simulink model "HorizontalBaseline"  (R2026b)
settings: Solver=FixedStepDiscrete  StopTime=inf  FixedStep=Official.Step
PostLoadFcn:
  | run(fullfile(fileparts(get_param('StampFly_IMU400','FileName')),'config','startup.m'));
InitFcn:
  | init_imu_flight;
undefined symbols (not defined in the file): Official
libraries: slpidlib x7, simulink x4, mspfiltlib x1
(part 1 of 5)
settings Model: SILPILModeSetting=veronly  Creator=tyasukaw  LastModifiedBy=tyasukaw
settings SolverCC: AutoInsertRateTranBlk=on
settings OptimizationCC: DifferentSizesBufferReuse=on  EfficientTunableParamExpr=on  EnhancedBackFolding=on  MaxStackSize=64  OptimizationCustomize=off  OptimizeBlockOrder=speed  PassReuseOutputArgsAs=Individual arguments  RemoveInternalMemoryZeroInit=on  RemoveRootLevelIOMemoryZeroInit=on
settings DebuggingCC: ParameterTunabilityLossMsg=error
settings HardwareCC: ProdHWDeviceType=ARM Compatible->ARM Cortex  ProdLargestAtomicFloat=Double  ProdLargestAtomicInteger=Long
settings SFSimCC: MATLABDynamicMemAlloc=off
settings RTWCC: BuildConfiguration=Faster Runs  DataTypeReplacement=CDataTypesFixedWidth  Description=Embedded Coder  HardwareBoard=ESP32-S3 Series (Arduino Compatible)  SystemTargetFile=ert.tlc  TLCOptions="-aInlineSetEventsForThisBaseRateFcn=TLC_FALSE -aSuppressMultiTaskScheduler=TLC_FALSE  -aRateBasedStepFcn=0"  TemplateMakefile=ert_default_tmf  Toolchain=ESP32
settings CodeAppCC: ForceParamTrailComments=on  IgnoreCustomStorageClasses=off  InsertBlockDesc=on  OperatorAnnotations=on  SFDataObjDesc=on  SimulinkDataObjDesc=on
settings ERTTargetCC: CombineSignalStateStructs=on  ExtModeAutomaticAllocSize=off  ExtModeIntrfLevel=Level2 - Open  ExtModeMexFile=ext_xcp  ExtModeStaticAlloc=on  MaxIdInt16=INT16_MAX  MaxIdInt32=INT32_MAX  MaxIdInt64=INT64_MAX  MaxIdInt8=INT8_MAX  MaxIdUint16=UINT16_MAX  MaxIdUint32=UINT32_MAX  MaxIdUint64=UINT64_MAX  MaxIdUint8=UINT8_MAX  MinIdInt16=INT16_MIN  MinIdInt32=INT32_MIN  MinIdInt64=INT64_MIN  MinIdInt8=INT8_MIN  SupportContinuousTime=on  SupportVariableSizeSignals=on

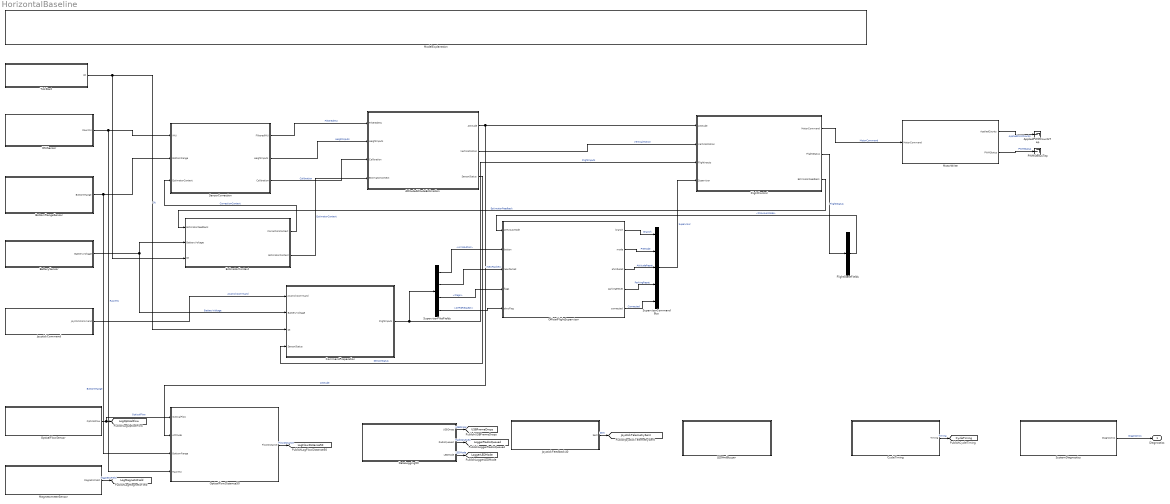
== system HorizontalBaseline ==
  AppliedPWMCountsTap : Terminator
      settings: Description=AppliedPWMCountsTap：使用しない観測出力をここで終端します。接続された制御信号を変更しません。
  AttitudeAltitudeEstimation : Subsystem  Description=IMU Filter で姿勢・補正済み角速度、MATLAB Function の AltitudeKalman で高度・鉛直速度を推定します。状態フラグと推定診断をまとめ、ログ用 Goto をこの階層から公開します。
      mask help: IMU Filter で姿勢・補正済み角速度、MATLAB Function の AltitudeKalman で高度・鉛直速度を推定します。状態フラグと推定診断をまとめ、ログ用 Goto をこの階層から公開します。
      mask Display: disp('AttitudeAltitudeEstimation');port_label('input',1,'FilteredIMU');port_label('input',2,'HeightInputs');port_label('input',3,'Calibration');port_label('input',4,'EstimatorContext');port_label('output',1,'Attitude');port_label('output',2,'VerticalMotion');port_label('output',3,'SensorStatus');
  BatterySensor : Subsystem  Description=電池電圧 [V] と読み出し有効性を取得します。I2C 使用中は前回値を保持し、ReadValid=0 を公開します。
      mask help: 電池電圧 [V] と読み出し有効性を取得します。I2C 使用中は前回値を保持し、ReadValid=0 を公開します。
      mask Display: disp('BatterySensor');port_label('output',1,'BatteryVoltage');
  BottomRangeSensor : Subsystem  Description=下向き ToF の初期化完了後は Mode に依存せず取得します。距離 [mm] と Fresh を BottomRange バスへまとめ、Status と診断は Goto で公開します。Fresh は 400 Hz の読み出しではなく新しい測定結果の到着を示します。前方センサーは未使用です。
      mask help: 下向き ToF の初期化完了後は Mode に依存せず取得します。距離 [mm] と Fresh を BottomRange バスへまとめ、Status と診断は Goto で公開します。Fresh は 400 Hz の読み出しではなく新しい測定結果の到着を示します。前方センサーは未使用です。
      mask Display: disp('BottomRangeSensor');port_label('output',1,'BottomRange');
  CommandPreparation : Subsystem  Description=操縦指令、電池電圧、実測 dt、センサーフラグを名前付きバスへまとめます。Stateflow と飛行制御へ同じ入力を渡し、ログ用の観測も公開します。
      mask help: 操縦指令、電池電圧、実測 dt、センサーフラグを名前付きバスへまとめます。Stateflow と飛行制御へ同じ入力を渡し、ログ用の観測も公開します。
      mask Display: disp('CommandPreparation');port_label('input',1,'JoystickCommand');port_label('input',2,'BatteryVoltage');port_label('input',3,'Dt');port_label('input',4,'SensorStatus');port_label('output',1,'FlightInputs');
  CycleTiming : Subsystem  Description=ログとモーター適用後の処理時間・周期間隔を観測します。制御値を変更せず、計測位置を信号依存で固定します。
      mask help: ログとモーター適用後の処理時間・周期間隔を観測します。制御値を変更せず、計測位置を信号依存で固定します。
      mask Display: disp('CycleTiming');port_label('output',1,'Timing');
  DataLogging50 : Subsystem  Description=生センサー・推定・制御・追加センサーを名前付き From で取得し、50 Hz の SFI8/SFIX/SFIY ログを生成して送信します。型・順序・CRC は維持します。Channel は RadioUSBTransport50 の設定画面で操縦側と揃えます。
      mask help: 生センサー・推定・制御・追加センサーを名前付き From で取得し、50 Hz の SFI8/SFIX/SFIY ログを生成して送信します。型・順序・CRC は維持します。Channel は RadioUSBTransport50 の設定画面で操縦側と揃えます。
      mask Display: disp('DataLogging50');port_label('output',1,'USBDrops');port_label('output',2,'RadioQueued');port_label('output',3,'LEDMode');
  EstimatorContext : Subsystem  Description=前周期のモード、高度制御許可、姿勢・待機リセットを 1 周期保持して推定器へ渡します。状態更新順序と代数ループ回避に必要な遅延です。
      mask help: 前周期のモード、高度制御許可、姿勢・待機リセットを 1 周期保持して推定器へ渡します。状態更新順序と代数ループ回避に必要な遅延です。
      mask Display: disp('EstimatorContext');port_label('input',1,'EstimatorFeedback');port_label('input',2,'BatteryVoltage');port_label('input',3,'Dt');port_label('output',1,'CorrectionContext');port_label('output',2,'EstimatorContext');
  FlightControl : Subsystem  Description=最上位 Stateflow の指令と姿勢・高度を受け、離着陸、7 個の PID、モーター配分を計算します。出力は Duty・PWM Counts、飛行状態、次周期の推定器コンテキストです。状態ログもこの階層に含みます。
      mask help: 最上位 Stateflow の指令と姿勢・高度を受け、離着陸、7 個の PID、モーター配分を計算します。出力は Duty・PWM Counts、飛行状態、次周期の推定器コンテキストです。状態ログもこの階層に含みます。
      mask Display: disp('FlightControl');port_label('input',1,'Attitude');port_label('input',2,'VerticalMotion');port_label('input',3,'FlightInputs');port_label('input',4,'Supervisor');port_label('output',1,'MotorCommand');port_label('output',2,'FlightStatus');port_label('output',3,'EstimatorFeedback');
  FlightStateFields : BusSelector  Description=FlightStateFields：バスから PreviousMode を選びます。元のベクトルの成分順序は変更しません。  OutputSignals=PreviousMode
  IMUSensor : Subsystem  Description=BMI270 の生加速度・角速度を XYZ のままバスへまとめます。センサー座標であり、単位は m/s²・rad/s。温度と Fresh は名前付き Goto でログへ公開します。
      mask help: BMI270 の生加速度・角速度を XYZ のままバスへまとめます。センサー座標であり、単位は m/s²・rad/s。温度と Fresh は名前付き Goto でログへ公開します。
      mask Display: disp('IMUSensor');port_label('output',1,'RawIMU');
  JoystickCommand : Subsystem  Description=公式 JoyStick から通常飛行の指令を受信し、操縦バスと診断を公開します。Flip 用押し込みボタンは使用しません。専用 Channel は内部の BasicJoystick で設定します。
      mask help: 公式 JoyStick から通常飛行の指令を受信し、操縦バスと診断を公開します。Flip 用押し込みボタンは使用しません。専用 Channel は内部の BasicJoystick で設定します。
      mask Display: disp('JoystickCommand');port_label('output',1,'JoystickCommand');
  JoystickFeedback40 : Subsystem  Description=公式 JoyStick の画面へ姿勢・高度・電池・制御状態を 40 Hz で返信します。通常ログとは別の公式 120 byte 形式です。
      mask help: 公式 JoyStick の画面へ姿勢・高度・電池・制御状態を 40 Hz で返信します。通常ログとは別の公式 120 byte 形式です。
      mask Display: disp('JoystickFeedback40');port_label('output',1,'Sent');
  LEDAndBuzzer : Subsystem  Description=飛行状態・電池・通信・姿勢リセット要求から LED と音を決め、出力キューへ渡します。機体ボタンの押下・解放による再起動もここで扱います。
      mask help: 飛行状態・電池・通信・姿勢リセット要求から LED と音を決め、出力キューへ渡します。機体ボタンの押下・解放による再起動もここで扱います。
      mask Display: disp('LEDAndBuzzer');
  MagnetometerSensor : Subsystem  Description=BMM150 の磁場 XYZ [μT] と有効性・Fresh・診断を取得します。センサー座標を保ってログへ渡し、姿勢推定・制御には使いません。
      mask help: BMM150 の磁場 XYZ [μT] と有効性・Fresh・診断を取得します。センサー座標を保ってログへ渡し、姿勢推定・制御には使いません。
      mask Display: disp('MagnetometerSensor');port_label('output',1,'MagneticField');
  ModelExplanation : Subsystem  Description=StampFly の学習用実装。400 Hz でセンサー取得→校正→姿勢・高度推定→離着陸と 7 PID→4 モーターへ処理します。Flip はありません。最上位 Stateflow がモードを管理し、下段は観測・記録・状態表示です。
      mask help: StampFly の学習用実装。400 Hz でセンサー取得→校正→姿勢・高度推定→離着陸と 7 PID→4 モーターへ処理します。Flip はありません。最上位 Stateflow がモードを管理し、下段は観測・記録・状態表示です。
      mask Display: disp(sprintf('StampFly IMU Filter / 400 Hz\nセンサー取得 → 校正・前処理 → 姿勢・高度推定 → PID → モーター\n飛行モードは最上位のStateflowで管理。下段は観測・記録・状態表示。'));
  MotorWrite : Subsystem  Description=8 bit の Counts を実機モーターへ適用します。順序 [FR, FL, RR, RL]、GPIO [42, 5, 41, 10]、150 kHz 指定です。実適用 Counts と PWM 診断を Goto で公開します。
      mask help: 8 bit の Counts を実機モーターへ適用します。順序 [FR, FL, RR, RL]、GPIO [42, 5, 41, 10]、150 kHz 指定です。実適用 Counts と PWM 診断を Goto で公開します。
      mask Display: disp('MotorWrite');port_label('input',1,'MotorCommand');port_label('output',1,'AppliedCounts');port_label('output',2,'PWMStatus');
  OfficialFlightSupervisor : Stateflow chart  Description=最上位の飛行状態管理です。前周期 Mode、操縦ボタン、新パケット、異常フラグ、姿勢リセットを受け、校正・待機・飛行・着陸の分岐と推定器リセットを決めます。  TreatAsAtomicUnit=on
      mask help: 最上位の飛行状態管理です。前周期 Mode、操縦ボタン、新パケット、異常フラグ、姿勢リセットを受け、校正・待機・飛行・着陸の分岐と推定器リセットを決めます。
  OpticalFlowDistance50 : Subsystem  Description=生の累積光学フロー、姿勢、角速度、下向き ToF から平面上の東・北移動距離を 50 Hz で作ります。回転補償と品質判定を行い、無効な区間は位置を保持します。385 count/rad は初期値です。
      mask help: 生の累積光学フロー、姿勢、角速度、下向き ToF から平面上の東・北移動距離を 50 Hz で作ります。回転補償と品質判定を行い、無効な区間は位置を保持します。385 count/rad は初期値です。
      mask Display: disp('OpticalFlowDistance50');port_label('input',1,'OpticalFlow');port_label('input',2,'Attitude');port_label('input',3,'BottomRange');port_label('input',4,'RawIMU');port_label('output',1,'FlowDistance');
  OpticalFlowSensor : Subsystem  Description=PMW3901 の生 2 軸差分・品質・診断・累積カウントを取得します。表示・記録専用で、水平位置制御へは戻しません。
      mask help: PMW3901 の生 2 軸差分・品質・診断・累積カウントを取得します。表示・記録専用で、水平位置制御へは戻しません。
      mask Display: disp('OpticalFlowSensor');port_label('output',1,'OpticalFlow');
  PWMStatusTap : Terminator
      settings: Description=PWMStatusTap：使用しない観測出力をここで終端します。接続された制御信号を変更しません。
  SensorCorrection : Subsystem  Description=センサー座標から機体 XYZ へ変換し、800 周期の静止校正とフィルターを行います。加速度 XYZ・角速度 XYZ の順を維持し、ToF の保持・外れ値処理と鉛直加速度もまとめます。推定用の前処理は Mode 0, 1 で保持します。
      mask help: センサー座標から機体 XYZ へ変換し、800 周期の静止校正とフィルターを行います。加速度 XYZ・角速度 XYZ の順を維持し、ToF の保持・外れ値処理と鉛直加速度もまとめます。推定用の前処理は Mode 0, 1 で保持します。
      mask Display: disp('SensorCorrection');port_label('input',1,'IMU');port_label('input',2,'BottomRange');port_label('input',3,'EstimatorContext');port_label('output',1,'FilteredIMU');port_label('output',2,'HeightInputs');port_label('output',3,'Calibration');
  SupervisorCommandBus : BusCreator  Description=SupervisorCommandBus：異なる単位・型を持つ関連信号を名前付きバスにまとめます。入力線の信号名が項目名です。  Inputs=5
  SupervisorPilotFields : BusSelector  Description=SupervisorPilotFields：バスから ArmButton,NewPacket,Flags,AHRSRequest を選びます。元のベクトルの成分順序は変更しません。  OutputSignals=ArmButton,NewPacket,Flags,AHRSRequest
  SystemDiagnostics : Subsystem  Description=各機能の診断 From を型付き名前付きバスへまとめます。50 Hz/40 Hz の値を必要な箇所で保持し、全体の診断出力へ渡します。
      mask help: 各機能の診断 From を型付き名前付きバスへまとめます。50 Hz/40 Hz の値を必要な箇所で保持し、全体の診断出力へ渡します。
      mask Display: disp('SystemDiagnostics');port_label('output',1,'Diagnostics');
  TickStart : Subsystem  Description=400 Hz 周期の開始時刻、実測 dt、タイマー診断を取得し、秒への時刻変換と Goto 公開をこの階層でまとめます。
      mask help: 400 Hz 周期の開始時刻、実測 dt、タイマー診断を取得し、秒への時刻変換と Goto 公開をこの階層でまとめます。
      mask Display: disp('TickStart');port_label('output',1,'Dt');
  Diagnostics : Outport  OutDataTypeStr=Bus: OfficialDiagnosticBus  BusOutputAsStruct=on
  tag scope: CycleTiming=global, JoystickTelemetrySent=global, LogFlowDistance50=global, LogMagneticField=global, LogOpticalFlow=global, LoggerLEDMode=global, LoggerRadioQueued=global, USBFrameDrops=global
  wires:
  JoystickFeedback40/1(Sent) -> [JoystickTelemetrySent]  "Sent"
  CycleTiming/1(Timing) -> [CycleTiming]  "Timing"
  AttitudeAltitudeEstimation/2(VerticalMotion) -> FlightControl/2(VerticalMotion)  "VerticalMotion"
  SensorCorrection/1(FilteredIMU) -> AttitudeAltitudeEstimation/1(FilteredIMU)  "FilteredIMU"
  SensorCorrection/2(HeightInputs) -> AttitudeAltitudeEstimation/2(HeightInputs)  "HeightInputs"
  SensorCorrection/3(Calibration) -> AttitudeAltitudeEstimation/3(Calibration)  "Calibration"
  SystemDiagnostics/1(Diagnostics) -> Diagnostics/1  "Diagnostics"
  DataLogging50/1(USBDrops) -> [USBFrameDrops]  "USBDrops"
  DataLogging50/2(RadioQueued) -> [LoggerRadioQueued]  "RadioQueued"
  DataLogging50/3(LEDMode) -> [LoggerLEDMode]  "LEDMode"
  SupervisorCommandBus/1 -> FlightControl/4(Supervisor)  "Supervisor"
  OfficialFlightSupervisor/5(connected) -> SupervisorCommandBus/5  "Connected"
  OfficialFlightSupervisor/4(parkingReset) -> SupervisorCommandBus/4  "ParkingReset"
  OfficialFlightSupervisor/3(ahrsReset) -> SupervisorCommandBus/3  "AttitudeReset"
  OfficialFlightSupervisor/2(mode) -> SupervisorCommandBus/2  "PreMode"
  OfficialFlightSupervisor/1(branch) -> SupervisorCommandBus/1  "Branch"
  SupervisorPilotFields/4 -> OfficialFlightSupervisor/5(ahrsFlag)  "<AHRSRequest>"
  SupervisorPilotFields/3 -> OfficialFlightSupervisor/4(flags)  "<Flags>"
  SupervisorPilotFields/2 -> OfficialFlightSupervisor/3(newPacket)  "<NewPacket>"
  SupervisorPilotFields/1 -> OfficialFlightSupervisor/2(button)  "<ArmButton>"
  FlightStateFields/1 -> OfficialFlightSupervisor/1(previousMode)  "<PreviousMode>"
  FlightControl/2(FlightStatus) -> FlightStateFields/1  "FlightStatus"
  FlightControl/1(MotorCommand) -> MotorWrite/1(MotorCommand)  "MotorCommand"
  MotorWrite/1(AppliedCounts) -> AppliedPWMCountsTap/1  "AppliedPWMCounts"
  MotorWrite/2(PWMStatus) -> PWMStatusTap/1  "PWMStatus"
  AttitudeAltitudeEstimation/3(SensorStatus) -> CommandPreparation/4(SensorStatus)  "SensorStatus"
  CommandPreparation/1(FlightInputs) -> SupervisorPilotFields/1, FlightControl/3(FlightInputs)  "FlightInputs"
  TickStart/1(Dt) -> EstimatorContext/3(Dt), CommandPreparation/3(Dt)  "Dt"
  BatterySensor/1(BatteryVoltage) -> EstimatorContext/2(BatteryVoltage), CommandPreparation/2(BatteryVoltage)  "BatteryVoltage"
  JoystickCommand/1(JoystickCommand) -> CommandPreparation/1(JoystickCommand)  "JoystickCommand"
  EstimatorContext/1(CorrectionContext) -> SensorCorrection/3(EstimatorContext)  "CorrectionContext"
  FlightControl/3(EstimatorFeedback) -> EstimatorContext/1(EstimatorFeedback)  "EstimatorFeedback"
  EstimatorContext/2(EstimatorContext) -> AttitudeAltitudeEstimation/4(EstimatorContext)  "EstimatorContext"
  BottomRangeSensor/1(BottomRange) -> SensorCorrection/2(BottomRange), OpticalFlowDistance50/3(BottomRange)  "BottomRange"
  OpticalFlowSensor/1(OpticalFlow) -> [LogOpticalFlow], OpticalFlowDistance50/1(OpticalFlow)  "OpticalFlow"
  IMUSensor/1(RawIMU) -> OpticalFlowDistance50/4(RawIMU), SensorCorrection/1(IMU)  "RawIMU"
  AttitudeAltitudeEstimation/1(Attitude) -> FlightControl/1(Attitude), OpticalFlowDistance50/2(Attitude)  "Attitude"
  OpticalFlowDistance50/1(FlowDistance) -> [LogFlowDistance50]  "FlowDistance"
  MagnetometerSensor/1(MagneticField) -> [LogMagneticField]  "MagneticField"

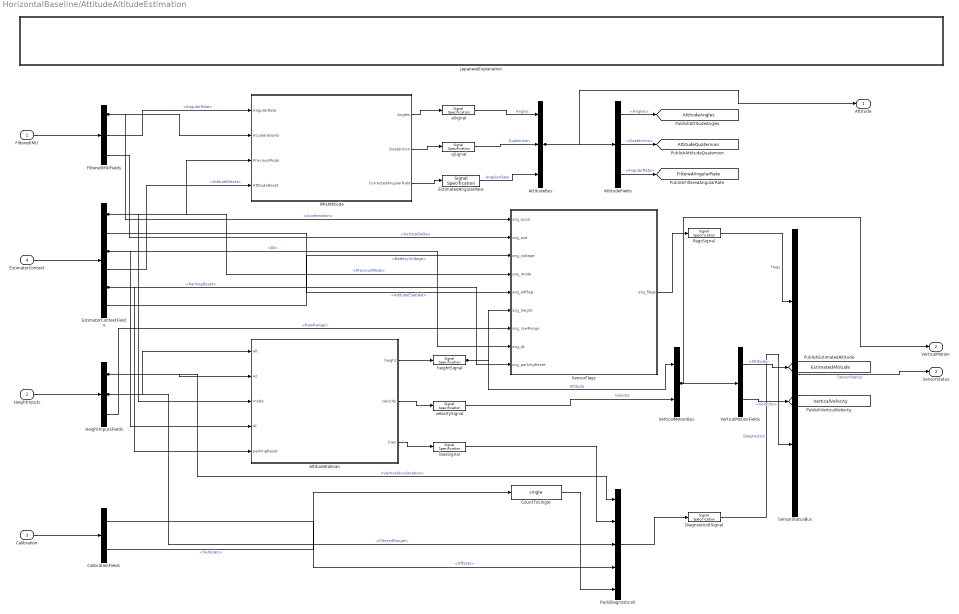
== system HorizontalBaseline/AttitudeAltitudeEstimation ==
  FilteredIMU : Inport
  HeightInputs : Inport  Port=2
  Calibration : Inport  Port=3
  EstimatorContext : Inport  Port=4
  AltitudeKalman : MATLAB Function  Description=下向き ToF の保持・平滑化した高さと鉛直加速度から、高度 [m]・鉛直速度・加速度バイアスを推定します。状態は [速度; 高度; バイアス]。公式実装の single 演算順序とリセット動作を保つ MATLAB Function です。加速度入力は従来どおり g 基準の数値です。  TreatAsAtomicUnit=on
  AttitudeBus : BusCreator  Description=AttitudeBus：異なる単位・型を持つ関連信号を名前付きバスにまとめます。入力線の信号名が項目名です。  Inputs=3
  AttitudeFields : BusSelector  Description=AttitudeFields：バスから Angles,Quaternion,AngularRate を選びます。元のベクトルの成分順序は変更しません。  OutputSignals=Angles,Quaternion,AngularRate
  CalibrationFields : BusSelector  Description=CalibrationFields：バスから Offsets,Samples を選びます。元のベクトルの成分順序は変更しません。  OutputSignals=Offsets,Samples
  CountToSingle : DataTypeConversion  Description=CountToSingle：後段のバス・演算に合わせて single 型へ変換します。  OutDataTypeStr=single  SaturateOnIntegerOverflow=off  RndMeth=Floor
  Diagnostics8Signal : SignalSpecification  OutDataTypeStr=single  Dimensions=8
  EstimatedAngularRate : SignalSpecification  OutDataTypeStr=single  Dimensions=3
  EstimatorContextFields : BusSelector  Description=EstimatorContextFields：バスから PreviousMode,AltitudeEnabled,Dt,AttitudeReset,ParkingReset,BatteryVoltage を選びます。元のベクトルの成分順序は変更しません。  OutputSignals=PreviousMode,AltitudeEnabled,Dt,AttitudeReset,ParkingReset,BatteryVoltage
  FilteredIMUFields : BusSelector  Description=FilteredIMUFields：バスから Acceleration,AngularRate,VerticalDelta を選びます。元のベクトルの成分順序は変更しません。  OutputSignals=Acceleration,AngularRate,VerticalDelta
  HeightInputsFields : BusSelector  Description=HeightInputsFields：バスから VerticalAcceleration,FilteredRange,RawRange を選びます。元のベクトルの成分順序は変更しません。  OutputSignals=VerticalAcceleration,FilteredRange,RawRange
  IMUAttitude : Subsystem  Description=機体 XYZ と推定器座標の変換、標準 IMU Filter、制御用の姿勢と角速度への変換をまとめます。停止中の保持と再開時リセットを行います。
      mask help: 機体 XYZ と推定器座標の変換、標準 IMU Filter、制御用の姿勢と角速度への変換をまとめます。停止中の保持と再開時リセットを行います。
      mask Display: disp('IMUAttitude');port_label('input',1,'AngularRate');port_label('input',2,'AccelerationG');port_label('input',3,'PreviousMode');port_label('input',4,'AttitudeReset');port_label('output',1,'Angles');port_label('output',2,'Quaternion');port_label('output',3,'CorrectedAngularRate');
  JapaneseExplanation : Subsystem  Description=IMU Filter で姿勢・補正済み角速度、MATLAB Function の AltitudeKalman で高度・鉛直速度を推定します。状態フラグと推定診断をまとめ、ログ用 Goto をこの階層から公開します。
      mask help: IMU Filter で姿勢・補正済み角速度、MATLAB Function の AltitudeKalman で高度・鉛直速度を推定します。状態フラグと推定診断をまとめ、ログ用 Goto をこの階層から公開します。
      mask Display: disp(sprintf('IMU Filter で姿勢・補正済み角速度、MATLAB Function の AltitudeKalman で高度・鉛直速度を推\n定します。\n状態フラグと推定診断をまとめ、ログ用 Goto をこの階層から公開します。'));
  PackDiagnostics8 : Mux  Description=PackDiagnostics8：同じ型の値を入力端子の順でベクトルに結合します。ログ仕様・モーター順に対応する結合は順序を保ちます。  Inputs=5
  SensorFlags : MATLAB Function  Description=推定・状態管理で使う [過大加速度; 距離異常の継続回数; 低電圧の継続回数] を uint8 で出力します。短い揺れを平滑化し、距離は最大 20 回、低電圧は最大 100 回まで数えます。  TreatAsAtomicUnit=on
  SensorStatusBus : BusCreator  Description=SensorStatusBus：異なる単位・型を持つ関連信号を名前付きバスにまとめます。入力線の信号名が項目名です。  Inputs=2
  VerticalMotionBus : BusCreator  Description=VerticalMotionBus：異なる単位・型を持つ関連信号を名前付きバスにまとめます。入力線の信号名が項目名です。  Inputs=2
  VerticalMotionFields : BusSelector  Description=VerticalMotionFields：バスから Altitude,Velocity を選びます。元のベクトルの成分順序は変更しません。  OutputSignals=Altitude,Velocity
  aSignal : SignalSpecification  OutDataTypeStr=single  Dimensions=3
  biasSignal : SignalSpecification  OutDataTypeStr=single  Dimensions=1
  flagsSignal : SignalSpecification  OutDataTypeStr=uint8  Dimensions=3
  heightSignal : SignalSpecification  OutDataTypeStr=single  Dimensions=1
  qSignal : SignalSpecification  OutDataTypeStr=single  Dimensions=4
  velocitySignal : SignalSpecification  OutDataTypeStr=single  Dimensions=1
  Attitude : Outport
  VerticalMotion : Outport  Port=2
  SensorStatus : Outport  Port=3
  tag scope: AttitudeAngles=global, AttitudeQuaternion=global, EstimatedAltitude=global, FilteredAngularRate=global, VerticalVelocity=global
  wires:
  PackDiagnostics8/1 -> Diagnostics8Signal/1
  EstimatorContext/1 -> EstimatorContextFields/1
  HeightInputs/1 -> HeightInputsFields/1
  Calibration/1 -> CalibrationFields/1
  FilteredIMU/1 -> FilteredIMUFields/1
  EstimatedAngularRate/1 -> AttitudeBus/3  "AngularRate"
  EstimatorContextFields/6 -> SensorFlags/3(arg_voltage)  "<BatteryVoltage>"
  FilteredIMUFields/2 -> IMUAttitude/1(AngularRate)  "<AngularRate>"
  EstimatorContextFields/2 -> SensorFlags/5(arg_altFlag)  "<AltitudeEnabled>"
  EstimatorContextFields/5 -> SensorFlags/9(arg_parkingReset), AltitudeKalman/5(parkingReset)  "<ParkingReset>"
  FilteredIMUFields/1 -> SensorFlags/1(arg_accel), IMUAttitude/2(AccelerationG)  "<Acceleration>"
  EstimatorContextFields/1 -> IMUAttitude/3(PreviousMode), AltitudeKalman/3(mode), SensorFlags/4(arg_mode)  "<PreviousMode>"
  EstimatorContextFields/3 -> SensorFlags/8(arg_dt), AltitudeKalman/4(dt)  "<Dt>"
  FilteredIMUFields/3 -> SensorFlags/2(arg_azd)  "<VerticalDelta>"
  EstimatorContextFields/4 -> IMUAttitude/4(AttitudeReset)  "<AttitudeReset>"
  IMUAttitude/1(Angles) -> aSignal/1
  HeightInputsFields/1 -> PackDiagnostics8/1, AltitudeKalman/2(az)  "<VerticalAcceleration>"
  IMUAttitude/2(Quaternion) -> qSignal/1
  HeightInputsFields/2 -> PackDiagnostics8/3, AltitudeKalman/1(alt)  "<FilteredRange>"
  IMUAttitude/3(CorrectedAngularRate) -> EstimatedAngularRate/1
  HeightInputsFields/3 -> SensorFlags/7(arg_rawRange)  "<RawRange>"
  AltitudeKalman/1(height) -> heightSignal/1
  AltitudeKalman/2(velocity) -> velocitySignal/1
  AltitudeKalman/3(bias) -> biasSignal/1
  AttitudeFields/2 -> [AttitudeQuaternion]  "<Quaternion>"
  CountToSingle/1 -> PackDiagnostics8/5
  CalibrationFields/1 -> PackDiagnostics8/4  "<Offsets>"
  AttitudeFields/3 -> [FilteredAngularRate]  "<AngularRate>"
  AttitudeBus/1 -> AttitudeFields/1, Attitude/1
  CalibrationFields/2 -> CountToSingle/1  "<Samples>"
  aSignal/1 -> AttitudeBus/1  "Angles"
  qSignal/1 -> AttitudeBus/2  "Quaternion"
  heightSignal/1 -> SensorFlags/6(arg_height), VerticalMotionBus/1  "Altitude"
  velocitySignal/1 -> VerticalMotionBus/2  "Velocity"
  VerticalMotionBus/1 -> VerticalMotionFields/1, VerticalMotion/1
  biasSignal/1 -> PackDiagnostics8/2
  SensorFlags/1(arg_flags) -> flagsSignal/1
  Diagnostics8Signal/1 -> SensorStatusBus/2  "Diagnostics"
  AttitudeFields/1 -> [AttitudeAngles]  "<Angles>"
  flagsSignal/1 -> SensorStatusBus/1  "Flags"
  VerticalMotionFields/1 -> [EstimatedAltitude]  "<Altitude>"
  VerticalMotionFields/2 -> [VerticalVelocity]  "<Velocity>"
  SensorStatusBus/1 -> SensorStatus/1  "SensorStatus"

== system HorizontalBaseline/BatterySensor ==
  Battery : MATLABSystem  Description=機体の電池電圧 [V] と今回の読み出し成功 ReadValid を出力します。ToF・磁気と I2C の排他制御を共有し、使用中は待たずに前回値を返します。SampleTime は制御周期 0.0025 秒です。  Priority=4  System=official.Battery400  SampleTime=Official.Step  SimulateUsing=Code generation
      mask Type: official.Battery400
  BatteryVoltage : Outport
  tag scope: BatteryReadValid=global, BatteryVoltage=global
  wires:
  Battery/2 -> [BatteryReadValid]  "BatteryValid"
  Battery/1 -> BatteryVoltage/1, [BatteryVoltage]  "BatteryVoltage"

== system HorizontalBaseline/BottomRangeSensor ==
  BottomRangeBus : BusCreator  Description=BottomRangeBus：異なる単位・型を持つ関連信号を名前付きバスにまとめます。入力線の信号名が項目名です。  Inputs=2
  BottomToFSource : MATLABSystem  Description=初期化完了後は飛行モードに依存せず距離を取得します。距離 [mm]、Fresh、未使用の前方距離、Status、Info を出力します。I2C 読み出しは core0 の非同期処理で、400 Hz の制御は待ちません。推定側の校正・待機条件は別に管理します。  Priority=3  System=official.BottomToFSource  SampleTime=Official.Step  SimulateUsing=Code generation
      mask Type: official.BottomToFSource
  JapaneseExplanation : Subsystem  Description=下向き ToF の初期化完了後は Mode に依存せず取得します。距離 [mm] と Fresh を BottomRange バスへまとめ、Status と診断は Goto で公開します。Fresh は 400 Hz の読み出しではなく新しい測定結果の到着を示します。前方センサーは未使用です。
      mask help: 下向き ToF の初期化完了後は Mode に依存せず取得します。距離 [mm] と Fresh を BottomRange バスへまとめ、Status と診断は Goto で公開します。Fresh は 400 Hz の読み出しではなく新しい測定結果の到着を示します。前方センサーは未使用です。
      mask Display: disp(sprintf('下向き ToF の初期化完了後は Mode に依存せず取得します。\n距離 [mm] と Fresh を BottomRange バスへまとめ、Status と診断は Goto で公開します。\nFresh は 400 Hz の読み出しではなく新しい測定結果の到着を示します。\n前方センサーは未使用です。'));
  BottomRange : Outport
  tag scope: BottomDistanceMm=global, BottomRangeFresh=global, BottomRangeStatus=global, BottomToFDiagnostics=global, UnusedFrontRangeMm=global
  wires:
  BottomRangeBus/1 -> BottomRange/1  "BottomRange"
  BottomToFSource/5 -> [BottomToFDiagnostics]  "Info"
  BottomToFSource/4 -> [BottomRangeStatus]  "Status"
  BottomToFSource/3 -> [UnusedFrontRangeMm]  "FrontDistanceMm"
  BottomToFSource/2 -> BottomRangeBus/2, [BottomRangeFresh]  "Fresh"
  BottomToFSource/1 -> [BottomDistanceMm], BottomRangeBus/1  "DistanceMm"

== system HorizontalBaseline/CommandPreparation ==
  JoystickCommand : Inport
  BatteryVoltage : Inport  Port=2
  Dt : Inport  Port=3
  SensorStatus : Inport  Port=4
  CommandTapBus : BusCreator  Description=CommandTapBus：異なる単位・型を持つ関連信号を名前付きバスにまとめます。入力線の信号名が項目名です。  Inputs=2
  CommandTapFields : BusSelector  Description=CommandTapFields：バスから Sticks,AHRSRequest を選びます。元のベクトルの成分順序は変更しません。  OutputSignals=Sticks,AHRSRequest
  ControlInputs : BusCreator  Description=ControlInputs：異なる単位・型を持つ関連信号を名前付きバスにまとめます。入力線の信号名が項目名です。  Inputs=7
  JapaneseExplanation : Subsystem  Description=操縦指令、電池電圧、実測 dt、センサーフラグを名前付きバスへまとめます。Stateflow と飛行制御へ同じ入力を渡し、ログ用の観測も公開します。
      mask help: 操縦指令、電池電圧、実測 dt、センサーフラグを名前付きバスへまとめます。Stateflow と飛行制御へ同じ入力を渡し、ログ用の観測も公開します。
      mask Display: disp(sprintf('操縦指令、電池電圧、実測 dt、センサーフラグを名前付きバスへまとめます。\nStateflow と飛行制御へ同じ入力を渡し、ログ用の観測も公開します。'));
  JoystickCommandFields : BusSelector  Description=JoystickCommandFields：バスから Sticks,ArmButton,NewPacket,AHRSRequest を選びます。元のベクトルの成分順序は変更しません。  OutputSignals=Sticks,ArmButton,NewPacket,AHRSRequest
  SensorStatusFields : BusSelector  Description=SensorStatusFields：バスから Flags,Diagnostics を選びます。元のベクトルの成分順序は変更しません。  OutputSignals=Flags,Diagnostics
  SensorTapBus : BusCreator  Description=SensorTapBus：異なる単位・型を持つ関連信号を名前付きバスにまとめます。入力線の信号名が項目名です。  Inputs=2
  SensorTapFields : BusSelector  Description=SensorTapFields：バスから Flags,Diagnostics を選びます。元のベクトルの成分順序は変更しません。  OutputSignals=Flags,Diagnostics
  FlightInputs : Outport
  tag scope: AttitudeResetRequest=global, JoystickSticks=global, SensorDiagnostics=global, SensorFlags=global
  wires:
  ControlInputs/1 -> FlightInputs/1  "FlightInputs"
  CommandTapBus/1 -> CommandTapFields/1  "CommandTap"
  Dt/1 -> ControlInputs/6
  BatteryVoltage/1 -> ControlInputs/5
  CommandTapFields/2 -> [AttitudeResetRequest]  "<AHRSRequest>"
  SensorStatus/1 -> SensorStatusFields/1
  JoystickCommand/1 -> JoystickCommandFields/1
  JoystickCommandFields/4 -> CommandTapBus/2, ControlInputs/4  "<AHRSRequest>"
  JoystickCommandFields/3 -> ControlInputs/3  "<NewPacket>"
  JoystickCommandFields/2 -> ControlInputs/2  "<ArmButton>"
  JoystickCommandFields/1 -> CommandTapBus/1, ControlInputs/1  "<Sticks>"
  SensorTapFields/1 -> [SensorFlags]  "<Flags>"
  SensorStatusFields/1 -> ControlInputs/7, SensorTapBus/1  "<Flags>"
  SensorTapFields/2 -> [SensorDiagnostics]  "<Diagnostics>"
  SensorStatusFields/2 -> SensorTapBus/2  "<Diagnostics>"
  SensorTapBus/1 -> SensorTapFields/1  "SensorTap"
  CommandTapFields/1 -> [JoystickSticks]  "<Sticks>"

== system HorizontalBaseline/CycleTiming ==
  TimingEnd : MATLABSystem  Description=周期開始時刻からこの地点までの時間・周期間隔・平均・最大・超過などを記録します。IMU の Fresh、実適用 PWM、ログへの信号依存で計測位置を固定しています。全タスクの処理時間は生成 step のラッパーが別途計測します。  Priority=10000  System=official.TimingEnd400  SampleTime=Official.Step  SimulateUsing=Code generation
      mask Type: official.TimingEnd400
  Timing : Outport
  wires:
  [AppliedPWMCounts] -> TimingEnd/3
  [IMUSampleFresh] -> TimingEnd/2
  [CycleStartUs] -> TimingEnd/1
  TimingEnd/1 -> Timing/1  "Timing"
  [USBFrameDrops] -> TimingEnd/5
  [PWMStatus] -> TimingEnd/4

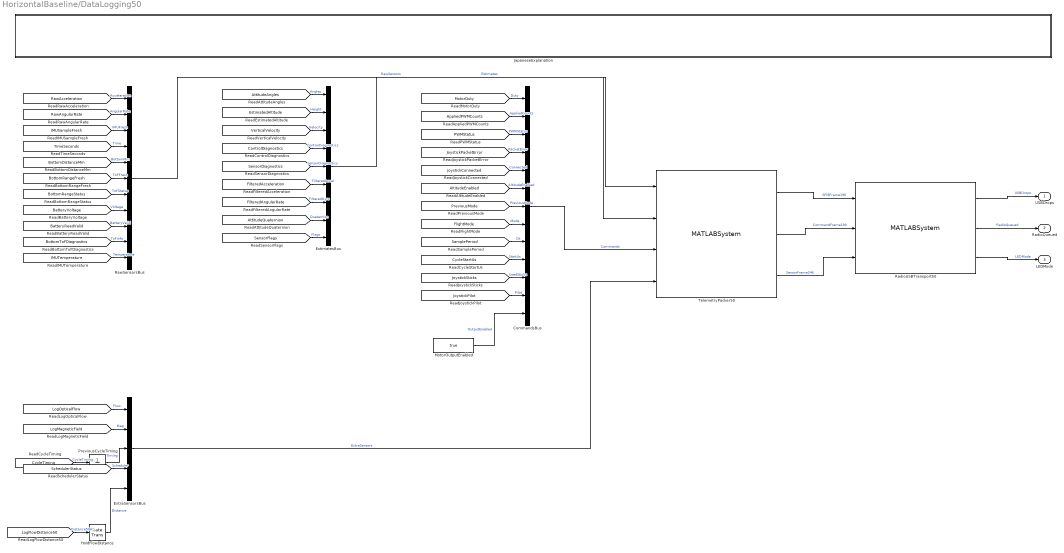
== system HorizontalBaseline/DataLogging50 ==
  CommandsBus : BusCreator  Description=CommandsBus：異なる単位・型を持つ関連信号を名前付きバスにまとめます。入力線の信号名が項目名です。  Inputs=13  OutDataTypeStr=Bus: BasicLogCommandBus  NonVirtualBus=on
  EstimatesBus : BusCreator  Description=EstimatesBus：異なる単位・型を持つ関連信号を名前付きバスにまとめます。入力線の信号名が項目名です。  Inputs=9  OutDataTypeStr=Bus: LogEstimateBus  NonVirtualBus=on
  ExtraSensorsBus : BusCreator  Description=ExtraSensorsBus：異なる単位・型を持つ関連信号を名前付きバスにまとめます。入力線の信号名が項目名です。  Inputs=5  OutDataTypeStr=Bus: LogExtraBus  NonVirtualBus=on
  HoldFlowDistance : RateTransition  OutPortSampleTime=.0025
  JapaneseExplanation : Subsystem  Description=生センサー・推定・制御・追加センサーを名前付き From で取得し、50 Hz の SFI8/SFIX/SFIY ログを生成して送信します。型・順序・CRC は維持します。Channel は RadioUSBTransport50 の設定画面で操縦側と揃えます。
      mask help: 生センサー・推定・制御・追加センサーを名前付き From で取得し、50 Hz の SFI8/SFIX/SFIY ログを生成して送信します。型・順序・CRC は維持します。Channel は RadioUSBTransport50 の設定画面で操縦側と揃えます。
      mask Display: disp(sprintf('生センサー・推定・制御・追加センサーを名前付き From で取得し、50 Hz の SFI8/SFIX/SFIY ログ\nを生成して送信します。\n型・順序・CRC は維持します。\nChannel は RadioUSBTransport50 の設定画面で操縦側と揃えます。'));
  MotorOutputEnabled : Constant  Description=MotorOutputEnabled：固定値 true を出力します。意味と単位は親の機能説明と信号名を参照します。  Value=true  OutDataTypeStr=boolean
  PreviousCycleTiming : UnitDelay  Description=PreviousCycleTiming：前周期の値を保持して出力します。更新順序と状態保持に必要な 1 周期遅延です。初期値 zeros(8,1,'uint32')、周期 .0025 秒。  InitialCondition=zeros(8,1,'uint32')  SampleTime=.0025
  RadioUSBTransport50 : MATLABSystem  Description=通常・操縦指令・追加センサーの 3 パケットを 50 Hz で ESP-NOW と USB の送信キューへ渡します。Queued はキュー投入成功、USBDrops は USB の欠落数です。到達は受信側で確認します。Channel を操縦指令受信ブロック・ログ受信機と同じ専用番号に設定します。  System=official.LogTransport50  Channel=uint8(3)  SimulateUsing=Code generation
      mask Type: official.LogTransport50
  RawSensorsBus : BusCreator  Description=RawSensorsBus：異なる単位・型を持つ関連信号を名前付きバスにまとめます。入力線の信号名が項目名です。  Inputs=11  OutDataTypeStr=Bus: LogRawBus  NonVirtualBus=on
  TelemetryPacker50 : MATLABSystem  Description=生センサー、推定、制御、追加センサーの名前付きバスを 50 Hz のログへ変換します。SFI8・SFIX・SFIY の項目順、型、CRC を保ちます。BuildID はプログラムの識別番号で、機体固有の ID ではありません。送信は後段の LogTransport50 が行います。  System=basic.ExtendedLogger50  BuildID=uint32( 1401 )  FirmwareRevision=uint32(1701)  SimulateUsing=Code generation
      mask Type: basic.ExtendedLogger50
  USBDrops : Outport
  RadioQueued : Outport  Port=2
  LEDMode : Outport  Port=3
  wires:
  [CycleStartUs] -> CommandsBus/10  "StartUs"
  [JoystickConnected] -> CommandsBus/5  "Connected"
  [FilteredAngularRate] -> EstimatesBus/7  "FilteredGyro"
  [BottomRangeFresh] -> RawSensorsBus/6  "ToFFresh"
  [FilteredAcceleration] -> EstimatesBus/6  "FilteredAccel"
  [ControlDiagnostics] -> EstimatesBus/4  "ControlDiagnostics"
  [IMUTemperature] -> RawSensorsBus/11  "Temperature"
  [BottomDistanceMm] -> RawSensorsBus/5  "BottomMm"
  [JoystickPilot] -> CommandsBus/12  "Pilot"
  [EstimatedAltitude] -> EstimatesBus/2  "Height"
  [BottomToFDiagnostics] -> RawSensorsBus/10  "ToFInfo"
  [IMUSampleFresh] -> RawSensorsBus/3  "IMUFresh"
  [FlightMode] -> CommandsBus/8  "Mode"
  [JoystickPacketError] -> CommandsBus/4  "PacketError"
  [BottomRangeStatus] -> RawSensorsBus/7  "ToFStatus"
  [CycleTiming] -> PreviousCycleTiming/1  "CycleTiming"
  [PWMStatus] -> CommandsBus/3  "PWMStatus"
  [TimeSeconds] -> RawSensorsBus/4  "Time"
  [JoystickSticks] -> CommandsBus/11  "UsedSticks"
  [RawAngularRate] -> RawSensorsBus/2  "AngularRate"
  CommandsBus/1 -> TelemetryPacker50/3  "Commands"
  [RawAcceleration] -> RawSensorsBus/1  "Acceleration"
  [SamplePeriod] -> CommandsBus/9  "Dt"
  [LogFlowDistance50] -> HoldFlowDistance/1  "Distance50Hz"
  [AppliedPWMCounts] -> CommandsBus/2  "AppliedCounts"
  [BatteryVoltage] -> RawSensorsBus/8  "Voltage"
  RadioUSBTransport50/2 -> RadioQueued/1  "RadioQueued"
  [AltitudeEnabled] -> CommandsBus/6  "AltitudeEnabled"
  [BatteryReadValid] -> RawSensorsBus/9  "BatteryValid"
  [AttitudeAngles] -> EstimatesBus/1  "Angles"
  [PreviousMode] -> CommandsBus/7  "PreviousMode"
  [VerticalVelocity] -> EstimatesBus/3  "Velocity"
  [LogOpticalFlow] -> ExtraSensorsBus/1  "Flow"
  [SensorDiagnostics] -> EstimatesBus/5  "SensorDiagnostics"
  [AttitudeQuaternion] -> EstimatesBus/8  "Quaternion"
  [MotorDuty] -> CommandsBus/1  "Duty"
  [SensorFlags] -> EstimatesBus/9  "Flags"
  MotorOutputEnabled/1 -> CommandsBus/13  "OutputEnabled"
  TelemetryPacker50/3 -> RadioUSBTransport50/3  "SensorFrame246"
  [SchedulerStatus] -> ExtraSensorsBus/4  "Scheduler"
  [LogMagneticField] -> ExtraSensorsBus/2  "Mag"
  PreviousCycleTiming/1 -> ExtraSensorsBus/3  "Timing"
  HoldFlowDistance/1 -> ExtraSensorsBus/5  "Distance"
  RawSensorsBus/1 -> TelemetryPacker50/1  "RawSensors"
  EstimatesBus/1 -> TelemetryPacker50/2  "Estimates"
  ExtraSensorsBus/1 -> TelemetryPacker50/4  "ExtraSensors"
  TelemetryPacker50/1 -> RadioUSBTransport50/1  "SFI8Frame190"
  TelemetryPacker50/2 -> RadioUSBTransport50/2  "CommandFrame190"
  RadioUSBTransport50/1 -> USBDrops/1  "USBDrops"
  RadioUSBTransport50/3 -> LEDMode/1  "LEDMode"

== system HorizontalBaseline/EstimatorContext ==
  EstimatorFeedback : Inport
  BatteryVoltage : Inport  Port=2
  Dt : Inport  Port=3
  CorrectionContextInternal : BusCreator  Description=CorrectionContextInternal：異なる単位・型を持つ関連信号を名前付きバスにまとめます。入力線の信号名が項目名です。  Inputs=2
  EstimatorContextInternal : BusCreator  Description=EstimatorContextInternal：異なる単位・型を持つ関連信号を名前付きバスにまとめます。入力線の信号名が項目名です。  Inputs=6
  EstimatorFeedbackFields : BusSelector  Description=EstimatorFeedbackFields：バスから PreviousMode,AltitudeEnabled,AttitudeReset,ParkingReset を選びます。元のベクトルの成分順序は変更しません。  OutputSignals=PreviousMode,AltitudeEnabled,AttitudeReset,ParkingReset
  JapaneseExplanation : Subsystem  Description=前周期のモード、高度制御許可、姿勢・待機リセットを 1 周期保持して推定器へ渡します。状態更新順序と代数ループ回避に必要な遅延です。
      mask help: 前周期のモード、高度制御許可、姿勢・待機リセットを 1 周期保持して推定器へ渡します。状態更新順序と代数ループ回避に必要な遅延です。
      mask Display: disp(sprintf('前周期のモード、高度制御許可、姿勢・待機リセットを 1 周期保持して推定器へ渡します。\n状態更新順序と代数ループ回避に必要な遅延です。'));
  CorrectionContext : Outport
  EstimatorContext : Outport  Port=2
  wires:
  CorrectionContextInternal/1 -> CorrectionContext/1  "CorrectionContext"
  BatteryVoltage/1 -> EstimatorContextInternal/6
  EstimatorFeedbackFields/4 -> EstimatorContextInternal/5  "<ParkingReset>"
  Dt/1 -> CorrectionContextInternal/2, EstimatorContextInternal/3
  EstimatorFeedbackFields/2 -> EstimatorContextInternal/2  "<AltitudeEnabled>"
  EstimatorFeedback/1 -> EstimatorFeedbackFields/1
  EstimatorFeedbackFields/3 -> EstimatorContextInternal/4  "<AttitudeReset>"
  EstimatorFeedbackFields/1 -> EstimatorContextInternal/1, CorrectionContextInternal/1  "<PreviousMode>"
  EstimatorContextInternal/1 -> EstimatorContext/1  "EstimatorContext"

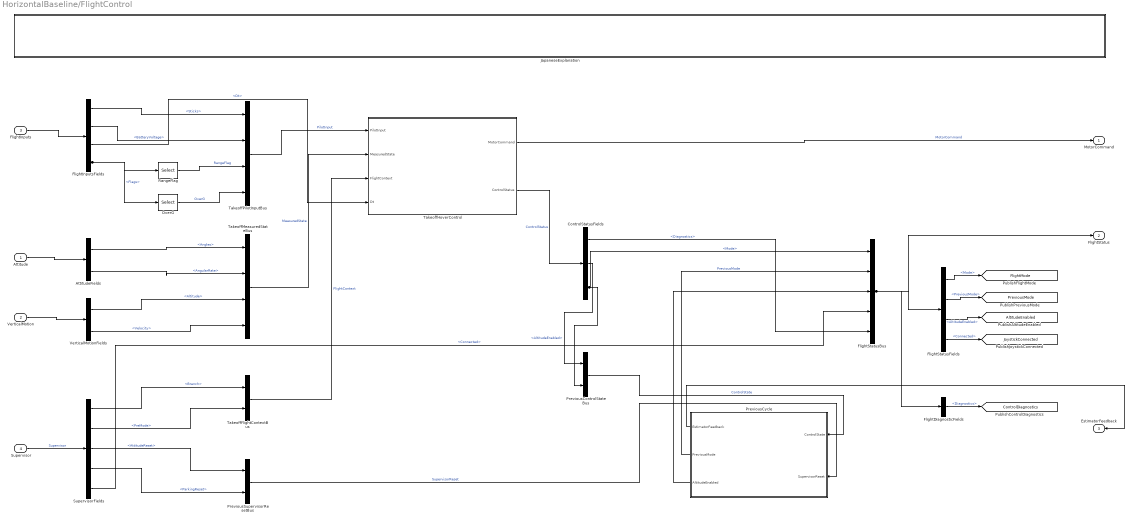
== system HorizontalBaseline/FlightControl ==
  Attitude : Inport
  VerticalMotion : Inport  Port=2
  FlightInputs : Inport  Port=3
  Supervisor : Inport  Port=4
  AttitudeFields : BusSelector  Description=AttitudeFields：バスから Angles,AngularRate を選びます。元のベクトルの成分順序は変更しません。  OutputSignals=Angles,AngularRate
  ControlStatusFields : BusSelector  Description=ControlStatusFields：バスから Diagnostics,AltitudeEnabled,Mode を選びます。元のベクトルの成分順序は変更しません。  OutputSignals=Diagnostics,AltitudeEnabled,Mode
  FlightDiagnosticFields : BusSelector  Description=FlightDiagnosticFields：バスから Diagnostics を選びます。元のベクトルの成分順序は変更しません。  OutputSignals=Diagnostics
  FlightInputsFields : BusSelector  Description=FlightInputsFields：バスから Sticks,BatteryVoltage,Dt,Flags を選びます。元のベクトルの成分順序は変更しません。  OutputSignals=Sticks,BatteryVoltage,Dt,Flags
  FlightStatusBus : BusCreator  Description=FlightStatusBus：異なる単位・型を持つ関連信号を名前付きバスにまとめます。入力線の信号名が項目名です。  Inputs=5
  FlightStatusFields : BusSelector  Description=FlightStatusFields：バスから Mode,PreviousMode,AltitudeEnabled,Connected を選びます。元のベクトルの成分順序は変更しません。  OutputSignals=Mode,PreviousMode,AltitudeEnabled,Connected
  JapaneseExplanation : Subsystem  Description=最上位 Stateflow の指令と姿勢・高度を受け、離着陸、7 個の PID、モーター配分を計算します。出力は Duty・PWM Counts、飛行状態、次周期の推定器コンテキストです。状態ログもこの階層に含みます。
      mask help: 最上位 Stateflow の指令と姿勢・高度を受け、離着陸、7 個の PID、モーター配分を計算します。出力は Duty・PWM Counts、飛行状態、次周期の推定器コンテキストです。状態ログもこの階層に含みます。
      mask Display: disp(sprintf('最上位 Stateflow の指令と姿勢・高度を受け、離着陸、7 個の PID、モーター配分を計算します。\n出力は Duty・PWM Counts、飛行状態、次周期の推定器コンテキストです。\n状態ログもこの階層に含みます。'));
  OverG : Selector  Description=OverG：必要なベクトル成分を選びます。選択位置は設定画面の Indices で確認します。  InputPortWidth=3  IndexOptions=Index vector (dialog)  Indices=1  OutputSizes=1
  PreviousControlStateBus : BusCreator  Description=PreviousControlStateBus：異なる単位・型を持つ関連信号を名前付きバスにまとめます。入力線の信号名が項目名です。  Inputs=2
  PreviousCycle : Subsystem  Description=前周期の推力・指令・モードなどを保持し、制御と次周期フィードバックへ渡します。Unit Delay は既存の更新順序を保つために必要です。
      mask help: 前周期の推力・指令・モードなどを保持し、制御と次周期フィードバックへ渡します。Unit Delay は既存の更新順序を保つために必要です。
      mask Display: disp('PreviousCycle');port_label('input',1,'ControlState');port_label('input',2,'SupervisorReset');port_label('output',1,'EstimatorFeedback');port_label('output',2,'PreviousMode');port_label('output',3,'AltitudeEnabled');
  PreviousSupervisorResetBus : BusCreator  Description=PreviousSupervisorResetBus：異なる単位・型を持つ関連信号を名前付きバスにまとめます。入力線の信号名が項目名です。  Inputs=2
  RangeFlag : Selector  Description=RangeFlag：必要なベクトル成分を選びます。選択位置は設定画面の Indices で確認します。  InputPortWidth=3  IndexOptions=Index vector (dialog)  Indices=2  OutputSizes=1
  SupervisorFields : BusSelector  Description=SupervisorFields：バスから Branch,PreMode,AttitudeReset,ParkingReset,Connected を選びます。元のベクトルの成分順序は変更しません。  OutputSignals=Branch,PreMode,AttitudeReset,ParkingReset,Connected
  TakeoffFlightContextBus : BusCreator  Description=TakeoffFlightContextBus：異なる単位・型を持つ関連信号を名前付きバスにまとめます。入力線の信号名が項目名です。  Inputs=2
  TakeoffHoverControl : Subsystem  Description=離着陸・高度制御・姿勢制御・角速度制御・モーター配分を機能別にまとめます。高度→速度、角度→角速度の二重ループを読みます。
      mask help: 離着陸・高度制御・姿勢制御・角速度制御・モーター配分を機能別にまとめます。高度→速度、角度→角速度の二重ループを読みます。
      mask Display: disp('TakeoffHoverControl');port_label('input',1,'PilotInput');port_label('input',2,'MeasuredState');port_label('input',3,'FlightContext');port_label('input',4,'Dt');port_label('output',1,'MotorCommand');port_label('output',2,'ControlStatus');
  TakeoffMeasuredStateBus : BusCreator  Description=TakeoffMeasuredStateBus：異なる単位・型を持つ関連信号を名前付きバスにまとめます。入力線の信号名が項目名です。  Inputs=4
  TakeoffPilotInputBus : BusCreator  Description=TakeoffPilotInputBus：異なる単位・型を持つ関連信号を名前付きバスにまとめます。入力線の信号名が項目名です。  Inputs=4
  VerticalMotionFields : BusSelector  Description=VerticalMotionFields：バスから Altitude,Velocity を選びます。元のベクトルの成分順序は変更しません。  OutputSignals=Altitude,Velocity
  MotorCommand : Outport
  FlightStatus : Outport  Port=2
  EstimatorFeedback : Outport  Port=3
  tag scope: AltitudeEnabled=global, ControlDiagnostics=global, FlightMode=global, JoystickConnected=global, PreviousMode=global
  wires:
  FlightInputsFields/2 -> TakeoffPilotInputBus/2  "<BatteryVoltage>"
  Supervisor/1 -> SupervisorFields/1  "Supervisor"
  FlightDiagnosticFields/1 -> [ControlDiagnostics]  "<Diagnostics>"
  FlightStatusFields/1 -> [FlightMode]  "<Mode>"
  TakeoffMeasuredStateBus/1 -> TakeoffHoverControl/2(MeasuredState)  "MeasuredState"
  VerticalMotion/1 -> VerticalMotionFields/1
  Attitude/1 -> AttitudeFields/1
  FlightInputsFields/4 -> RangeFlag/1, OverG/1  "<Flags>"
  FlightStatusFields/3 -> [AltitudeEnabled]  "<AltitudeEnabled>"
  FlightInputs/1 -> FlightInputsFields/1
  TakeoffPilotInputBus/1 -> TakeoffHoverControl/1(PilotInput)  "PilotInput"
  FlightInputsFields/3 -> TakeoffHoverControl/4(Dt)  "<Dt>"
  FlightStatusFields/4 -> [JoystickConnected]  "<Connected>"
  FlightInputsFields/1 -> TakeoffPilotInputBus/1  "<Sticks>"
  RangeFlag/1 -> TakeoffPilotInputBus/3  "RangeFlag"
  OverG/1 -> TakeoffPilotInputBus/4  "OverG"
  AttitudeFields/1 -> TakeoffMeasuredStateBus/1  "<Angles>"
  AttitudeFields/2 -> TakeoffMeasuredStateBus/2  "<AngularRate>"
  VerticalMotionFields/1 -> TakeoffMeasuredStateBus/3  "<Altitude>"
  VerticalMotionFields/2 -> TakeoffMeasuredStateBus/4  "<Velocity>"
  SupervisorFields/1 -> TakeoffFlightContextBus/1  "<Branch>"
  SupervisorFields/2 -> TakeoffFlightContextBus/2  "<PreMode>"
  PreviousSupervisorResetBus/1 -> PreviousCycle/2(SupervisorReset)  "SupervisorReset"
  SupervisorFields/3 -> PreviousSupervisorResetBus/1  "<AttitudeReset>"
  SupervisorFields/4 -> PreviousSupervisorResetBus/2  "<ParkingReset>"
  SupervisorFields/5 -> FlightStatusBus/4  "<Connected>"
  TakeoffFlightContextBus/1 -> TakeoffHoverControl/3(FlightContext)  "FlightContext"
  TakeoffHoverControl/1(MotorCommand) -> MotorCommand/1  "MotorCommand"
  TakeoffHoverControl/2(ControlStatus) -> ControlStatusFields/1  "ControlStatus"
  ControlStatusFields/1 -> FlightStatusBus/5  "<Diagnostics>"
  FlightStatusBus/1 -> FlightStatus/1, FlightStatusFields/1, FlightDiagnosticFields/1
  ControlStatusFields/2 -> PreviousControlStateBus/1  "<AltitudeEnabled>"
  ControlStatusFields/3 -> PreviousControlStateBus/2, FlightStatusBus/1  "<Mode>"
  PreviousCycle/3(AltitudeEnabled) -> FlightStatusBus/3
  PreviousCycle/2(PreviousMode) -> FlightStatusBus/2  "PreviousMode"
  PreviousCycle/1(EstimatorFeedback) -> EstimatorFeedback/1
  FlightStatusFields/2 -> [PreviousMode]  "<PreviousMode>"
  PreviousControlStateBus/1 -> PreviousCycle/1(ControlState)  "ControlState"

== system HorizontalBaseline/IMUSensor ==
  BMI270 : MATLABSystem  Description=SPI 接続の加速度 [m/s²]、角速度 [rad/s]、温度 [°C]、新規サンプル Status を出力します。XYZ はセンサー座標です。機体座標への変換は後段で行います。ODR は 400 Hz、レンジは ±8 g・±2000 deg/s。PC シミュレーションは 0 を返すため、検証には再生入力を使います。  Priority=2  System=stampfly.BMI270IMU  SampleTime=Official.Step  SimulateUsing=Code generation
      mask Type: stampfly.BMI270IMU
  JapaneseExplanation : Subsystem  Description=BMI270 の生加速度・角速度を XYZ のままバスへまとめます。センサー座標であり、単位は m/s²・rad/s。温度と Fresh は名前付き Goto でログへ公開します。
      mask help: BMI270 の生加速度・角速度を XYZ のままバスへまとめます。センサー座標であり、単位は m/s²・rad/s。温度と Fresh は名前付き Goto でログへ公開します。
      mask Display: disp(sprintf('BMI270 の生加速度・角速度を XYZ のままバスへまとめます。\nセンサー座標であり、単位は m/s²・rad/s。\n温度と Fresh は名前付き Goto でログへ公開します。'));
  RawIMUInternal : BusCreator  Description=RawIMUInternal：異なる単位・型を持つ関連信号を名前付きバスにまとめます。入力線の信号名が項目名です。  Inputs=2
  RawIMU : Outport
  tag scope: IMUSampleFresh=global, IMUTemperature=global, RawAcceleration=global, RawAngularRate=global
  wires:
  BMI270/1 -> RawIMUInternal/1, [RawAcceleration]  "Acceleration"
  BMI270/2 -> RawIMUInternal/2, [RawAngularRate]  "AngularRate"
  RawIMUInternal/1 -> RawIMU/1  "RawIMU"
  BMI270/3 -> [IMUTemperature]  "Temperature"
  BMI270/4 -> [IMUSampleFresh]  "IMUFresh"

== system HorizontalBaseline/JoystickCommand ==
  BasicJoystick : MATLABSystem  Description=公式 Atom JoyStick の指令を ESP-NOW で受信します。Stick6 は [Roll, Pitch, Yaw, Thrust, 制御モード, 高度モード]。アーム、通信状態、姿勢リセット、新パケット、エラーも出力します。Flip 用ボタンは無視します。Channel は自分専用の 1～13 にし、機体のログ送信・受信機と揃えます。  Priority=5  System=basic.Joystick400  SampleTime=.0025  Channel=uint8( 3 )  SimulateUsing=Code generation
      mask Type: basic.Joystick400
  JoystickCommandBus : BusCreator  Description=JoystickCommandBus：異なる単位・型を持つ関連信号を名前付きバスにまとめます。入力線の信号名が項目名です。  Inputs=4  OutDataTypeStr=Bus: BasicLogPilotBus  NonVirtualBus=on
  RadioDiagnosticsBus : BusCreator  Description=RadioDiagnosticsBus：異なる単位・型を持つ関連信号を名前付きバスにまとめます。入力線の信号名が項目名です。  Inputs=2
  RadioDiagnosticsFields : BusSelector  Description=RadioDiagnosticsFields：バスから LinkAge,PacketError を選びます。元のベクトルの成分順序は変更しません。  OutputSignals=LinkAge,PacketError
  RawRadioAgeUnused : Terminator
      settings: Description=RawRadioAgeUnused：使用しない観測出力をここで終端します。接続された制御信号を変更しません。
  JoystickCommand : Outport
  tag scope: JoystickPacketError=global, JoystickPilot=global
  wires:
  RadioDiagnosticsBus/1 -> RadioDiagnosticsFields/1  "RadioDiagnostics"
  BasicJoystick/6 -> RadioDiagnosticsBus/2  "PacketError"
  BasicJoystick/1 -> JoystickCommandBus/1  "Sticks"
  BasicJoystick/5 -> JoystickCommandBus/3  "NewPacket"
  BasicJoystick/2 -> JoystickCommandBus/2  "ArmButton"
  BasicJoystick/3 -> RadioDiagnosticsBus/1  "LinkAge"
  JoystickCommandBus/1 -> JoystickCommand/1, [JoystickPilot]  "JoystickCommand"
  BasicJoystick/4 -> JoystickCommandBus/4  "AHRSRequest"
  RadioDiagnosticsFields/1 -> RawRadioAgeUnused/1  "<LinkAge>"
  RadioDiagnosticsFields/2 -> [JoystickPacketError]  "<PacketError>"

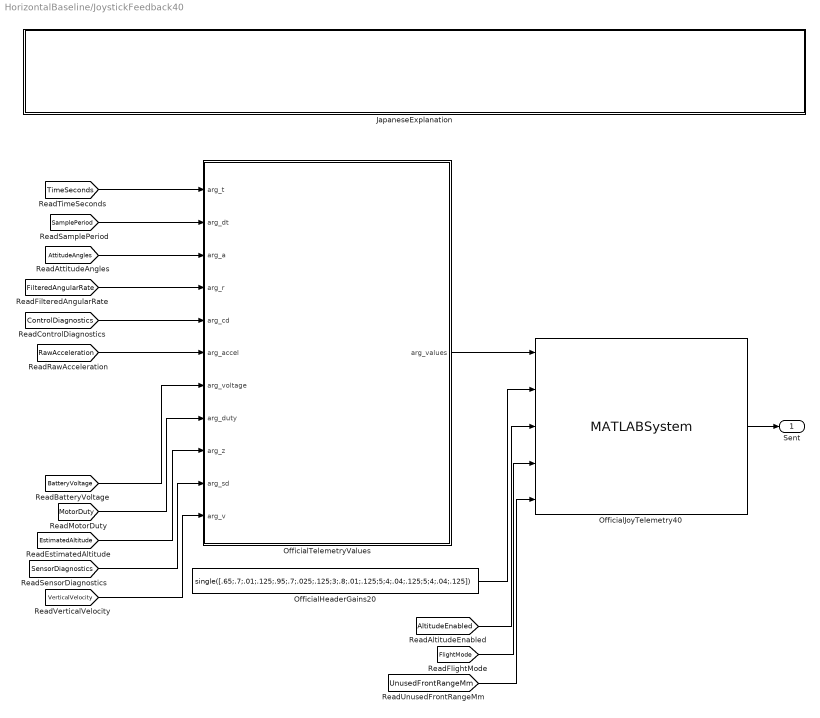
== system HorizontalBaseline/JoystickFeedback40 ==
  JapaneseExplanation : Subsystem  Description=公式 JoyStick の画面へ姿勢・高度・電池・制御状態を 40 Hz で返信します。通常ログとは別の公式 120 byte 形式です。
      mask help: 公式 JoyStick の画面へ姿勢・高度・電池・制御状態を 40 Hz で返信します。通常ログとは別の公式 120 byte 形式です。
      mask Display: disp(sprintf('公式 JoyStick の画面へ姿勢・高度・電池・制御状態を 40 Hz で返信します。\n通常ログとは別の公式 120 byte 形式です。'));
  OfficialHeaderGains20 : Constant  Description=OfficialHeaderGains20：固定値 single([.65;.7;.01;.125;.95;.7;.025;.125;3;.8;.01;.125;5;4;.04;.125;5;4;.04;.125]) を出力します。意味と単位は親の機能説明と信号名を参照します。  Value=single([.65;.7;.01;.125;.95;.7;.025;.125;3;.8;.01;.125;5;4;.04;.125;5;4;.04;.125])
  OfficialJoyTelemetry40 : MATLABSystem  Description=公式の 27 float 値とゲイン表、高度モード、飛行モード、前方距離を 40 Hz で JoyStick へ返信します。公式 120 byte 形式を保ちます。Sent は送信要求の結果です。  Priority=240  System=official.RadioTelemetryWrite40  SimulateUsing=Code generation
      mask Type: official.RadioTelemetryWrite40
  OfficialTelemetryValues : MATLAB Function  Description=JoyStick へ返す公式 120 byte テレメトリの 27 個の float 値を作ります。時刻・姿勢・目標・電池・加速度・速度・高度などを公式の単位と順序へ変換します。送信は後段の専用 I/O ブロックが行います。  TreatAsAtomicUnit=on
  Sent : Outport
  wires:
  [MotorDuty] -> OfficialTelemetryValues/8(arg_duty)
  [ControlDiagnostics] -> OfficialTelemetryValues/5(arg_cd)
  [FilteredAngularRate] -> OfficialTelemetryValues/4(arg_r)
  [AttitudeAngles] -> OfficialTelemetryValues/3(arg_a)
  [SamplePeriod] -> OfficialTelemetryValues/2(arg_dt)
  [TimeSeconds] -> OfficialTelemetryValues/1(arg_t)
  [BatteryVoltage] -> OfficialTelemetryValues/7(arg_voltage)
  [RawAcceleration] -> OfficialTelemetryValues/6(arg_accel)
  [EstimatedAltitude] -> OfficialTelemetryValues/9(arg_z)
  [SensorDiagnostics] -> OfficialTelemetryValues/10(arg_sd)
  [VerticalVelocity] -> OfficialTelemetryValues/11(arg_v)
  OfficialTelemetryValues/1(arg_values) -> OfficialJoyTelemetry40/1
  OfficialHeaderGains20/1 -> OfficialJoyTelemetry40/2
  [UnusedFrontRangeMm] -> OfficialJoyTelemetry40/5
  [AltitudeEnabled] -> OfficialJoyTelemetry40/3
  [FlightMode] -> OfficialJoyTelemetry40/4
  OfficialJoyTelemetry40/1 -> Sent/1

== system HorizontalBaseline/LEDAndBuzzer ==
  ControlMode : Selector  Description=ControlMode：必要なベクトル成分を選びます。選択位置は設定画面の Indices で確認します。  InputPortWidth=6  IndexOptions=Index vector (dialog)  Indices=5  OutputSizes=1
  LowVoltageCount : Selector  Description=LowVoltageCount：必要なベクトル成分を選びます。選択位置は設定画面の Indices で確認します。  InputPortWidth=3  IndexOptions=Index vector (dialog)  Indices=3  OutputSizes=1
  StatusIndicators : MATLAB Function  Description=飛行モード・電池・通信状態を LED 色とブザーへ変換します。待ち時間は 400 Hz のカウンターで管理し、機体ボタンの押下・解放を確認して再起動要求を出します。実際の LED・音・再起動は後段の I/O が行います。  TreatAsAtomicUnit=on
  StatusWrite : MATLABSystem  Description=RGB 色 2 個、ブザー周波数 [Hz]、再起動要求を機体の出力キューへ渡します。LED・音の更新は別タスクで実行します。再起動要求は機体の再起動に直結するので、状態判定ブロックからの信号を接続します。  System=official.StatusWrite400  SimulateUsing=Code generation
      mask Type: official.StatusWrite400
  UserButton : MATLABSystem  Description=StampS3 の GPIO0 ボタンを読み、押下中は uint8(1) を出力します。操縦用 JoyStick のボタンとは別です。押下時間と解放の判定は StatusIndicators で行います。  System=official.UserButton400  SimulateUsing=Code generation
      mask Type: official.UserButton400
  wires:
  [AttitudeResetRequest] -> StatusIndicators/6(arg_ahrsFlag)
  LowVoltageCount/1 -> StatusIndicators/4(arg_lowVoltage)
  [SensorFlags] -> LowVoltageCount/1
  [JoystickSticks] -> ControlMode/1
  [JoystickPacketError] -> StatusIndicators/5(arg_rcError)
  [AltitudeEnabled] -> StatusIndicators/3(arg_altFlag)
  [PreviousMode] -> StatusIndicators/1(arg_mode)
  ControlMode/1 -> StatusIndicators/2(arg_controlMode)
  UserButton/1 -> StatusIndicators/7(arg_button)
  StatusIndicators/1(arg_color1) -> StatusWrite/1
  StatusIndicators/2(arg_color2) -> StatusWrite/2
  StatusIndicators/3(arg_tone) -> StatusWrite/3
  StatusIndicators/4(arg_restart) -> StatusWrite/4

== system HorizontalBaseline/MagnetometerSensor ==
  DeviceRead : MATLABSystem  Description=BMM150 の補償済み磁場 XYZ [μT]、有効性・Fresh・エラー、診断を出力します。新規測定は約 30 Hz、モデルは 400 Hz で最新値を受け取ります。ToF・電池と I2C 排他を共有します。磁気は表示・記録用です。  System=stampfly.BMM150  I2CAddress=uint8( 16 )  SampleTime=.0025  SimulateUsing=Code generation
      mask Type: stampfly.BMM150
  JapaneseExplanation : Subsystem  Description=BMM150 の磁場 XYZ [μT] と有効性・Fresh・診断を取得します。センサー座標を保ってログへ渡し、姿勢推定・制御には使いません。
      mask help: BMM150 の磁場 XYZ [μT] と有効性・Fresh・診断を取得します。センサー座標を保ってログへ渡し、姿勢推定・制御には使いません。
      mask Display: disp(sprintf('BMM150 の磁場 XYZ [μT] と有効性・Fresh・診断を取得します。\nセンサー座標を保ってログへ渡し、姿勢推定・制御には使いません。'));
  SensorDataBus : BusCreator  Description=SensorDataBus：異なる単位・型を持つ関連信号を名前付きバスにまとめます。入力線の信号名が項目名です。  Inputs=3  OutDataTypeStr=Bus: LogMagBus  NonVirtualBus=on
  MagneticField : Outport
  wires:
  SensorDataBus/1 -> MagneticField/1  "SensorData"
  DeviceRead/1 -> SensorDataBus/1  "Field"
  DeviceRead/2 -> SensorDataBus/2  "Flags"
  DeviceRead/3 -> SensorDataBus/3  "Info"

== system HorizontalBaseline/ModelExplanation ==

== system HorizontalBaseline/MotorWrite ==
  MotorCommand : Inport
  JapaneseExplanation : Subsystem  Description=8 bit の Counts を実機モーターへ適用します。順序 [FR, FL, RR, RL]、GPIO [42, 5, 41, 10]、150 kHz 指定です。実適用 Counts と PWM 診断を Goto で公開します。
      mask help: 8 bit の Counts を実機モーターへ適用します。順序 [FR, FL, RR, RL]、GPIO [42, 5, 41, 10]、150 kHz 指定です。実適用 Counts と PWM 診断を Goto で公開します。
      mask Display: disp(sprintf('8 bit の Counts を実機モーターへ適用します。\n順序 [FR, FL, RR, RL]、GPIO [42, 5, 41, 10]、150 kHz 指定です。\n実適用 Counts と PWM 診断を Goto で公開します。'));
  MotorCommandFields : BusSelector  Description=MotorCommandFields：バスから Duty,Counts を選びます。元のベクトルの成分順序は変更しません。  OutputSignals=Duty,Counts
  MotorOutputEnabled : Constant  Description=MotorOutputEnabled：固定値 true を出力します。意味と単位は親の機能説明と信号名を参照します。  Value=true  SampleTime=Official.Step
  PWM150kHz8bit : MATLABSystem  Description=入力 Counts4 は [FR, FL, RR, RL] の 8 bit PWM カウントです。Enable と AllowMotorOutput が有効なとき実機へ適用し、実適用値と状態を返します。機体用は 150 kHz 指定です。これは回転数の測定値ではありません。  Priority=100  System=official.MotorPWM400  SampleTime=Official.Step  AllowMotorOutput=true  SimulateUsing=Code generation
      mask Type: official.MotorPWM400
  AppliedCounts : Outport
  PWMStatus : Outport  Port=2
  tag scope: AppliedPWMCounts=global, MotorDuty=global, PWMStatus=global
  wires:
  PWM150kHz8bit/2 -> [PWMStatus], PWMStatus/1
  MotorCommandFields/1 -> [MotorDuty]  "<Duty>"
  MotorCommand/1 -> MotorCommandFields/1
  MotorCommandFields/2 -> PWM150kHz8bit/1  "<Counts>"
  MotorOutputEnabled/1 -> PWM150kHz8bit/2
  PWM150kHz8bit/1 -> AppliedCounts/1, [AppliedPWMCounts]
